simulink library "AFCToolbox2023a"  (R2023a)
settings: Solver=VariableStepAuto  StartTime=0.0  StopTime=10.0  RelTol=1e-3
undefined symbols (not defined in the file or in its folder): AFC5Toolbox_SimuMoudle, AFCToolbox, ax, ay, az, btnSample, C_d, C_dm, C_m, C_t, Control, d, declination_table, dp0, dp1, dp2, dp3, dt, euler_0, g0, I_xyz, inclination_table, J_m, lmd_high, lmd_low, lp_acc_knoise, lp_acc_max, lp_acc_min, lp_acc_seed, lp_GPS_BL_max, lp_GPS_BL_min, lp_GPS_H_max, lp_GPS_H_min, lp_GPS_knoise, lp_GPS_seed, lp_GPS_vel_max, lp_GPS_vel_min, lp_gyro_knoise, lp_gyro_max, lp_gyro_min, lp_gyro_seed, lp_hf_vwind, lp_hs_vwind_interp, lp_kaerorho, lp_kaeroT, lp_kIxyz, lp_kmass, lp_momentx_A0, lp_momentx_Af, lp_momentx_ts, lp_momenty_A0, lp_momenty_Af, lp_momenty_ts, lp_momentz_A0, lp_momentz_Af, lp_momentz_ts, lp_vf_vwind, lp_vs_vwind_interp, lp_vwind_thetax, lp_vwind_thetaz ... (+54)
libraries: $bdroot x104, simulink x75, etargetslib x32, sharedtransform x13, simulink_extras x12, dspstat3 x11, aerolibconvert2 x9, aerolibtransform2 x3, aerolibutil x2, matrix_library x1
(part 4 of 10)

== system AFCToolbox2023a/SimuMoudle/Forces & Moments1/Moments ==
  w_xyz1 : Inport
  w_1234 : Inport  Port=2
  Abs : Abs  SaturateOnIntegerOverflow=off
  Constant : Constant  Value=[1 -1 -1 1;1 1 -1 -1]
  Constant1 : Constant  Value=[1 -1 1 -1]
  Constant2 : Constant  Value=[1 -1 1 -1]
  Constant3 : Constant  Value=[-1 1 -1 1]
  Constant4 : Constant  Value=0
  Disturb : Subsystem
  Dot Product : DotProduct  OutDataTypeStr=Inherit: Inherit via internal rule
  Dot Product1 : DotProduct  OutDataTypeStr=Inherit: Inherit via internal rule
  Dot Product2 : DotProduct  OutDataTypeStr=Inherit: Inherit via internal rule
  Gain : Gain  Gain=C_t
  Gain1 : Gain  Gain=d
  Gain2 : Gain  Gain=C_m
  Gain3 : Gain  Gain=C_dm
  Gain4 : Gain  Gain=-1
  Gain5 : Gain  Gain=J_m
  Gain6 : Gain  Gain=sqrt(2)/2
  M1 : Scope
  Mux : Mux  Inputs=2
  Mux1 : Mux  Inputs=3
  Product : Product  Multiplication=Matrix(*)
  Product{1,3,6..7} (4 alike) : Product
  Scope : Scope
  Selector : Selector  InputPortWidth=3  IndexOptions=Index vector (dialog)  Indices=2  OutputSizes=1
  Selector1 : Selector  InputPortWidth=3  IndexOptions=Index vector (dialog)  Indices=1  OutputSizes=1
  Subtract : Sum  Inputs=3
  Sum of Elements : Sum  Inputs=+
  Sum of Elements1 : Sum  Inputs=+
  M : Outport
  wires:
  Subtract/1 -> Disturb/1(Moment)
  Disturb/1(M) -> M/1, M1/1
  Product1/1 -> Gain2/1, Gain/1
  Gain/1 -> Gain1/1
  Constant/1 -> Gain6/1
  Gain1/1 -> Product/2
  Gain2/1 -> Dot Product2/2
  Constant1/1 -> Dot Product2/1
  Product/1 -> Mux/1
  Dot Product2/1 -> Mux/2
  Abs/1 -> Product3/2
  Product3/1 -> Gain3/1
  w_xyz1/1 -> Abs/1, Product3/1, Selector/1, Selector1/1
  Gain3/1 -> Gain4/1
  Constant2/1 -> Dot Product/1
  Constant3/1 -> Dot Product1/1
  Selector/1 -> Product6/2
  Dot Product/1 -> Sum of Elements/1
  Sum of Elements/1 -> Product6/1
  Dot Product1/1 -> Sum of Elements1/1
  Selector1/1 -> Product7/2
  Sum of Elements1/1 -> Product7/1
  Product6/1 -> Mux1/1
  Product7/1 -> Mux1/2
  Constant4/1 -> Mux1/3
  Mux1/1 -> Gain5/1
  Gain4/1 -> Subtract/1
  Mux/1 -> Subtract/2
  Gain6/1 -> Product/1
  w_1234/1 -> Scope/1, Product1/2, Product1/1, Dot Product1/2, Dot Product/2
  Gain5/1 -> Subtract/3

== system AFCToolbox2023a/SimuMoudle/Forces & Moments1/Parameters ==
  V_xyz : Inport
  xyz : Inport  Port=2
  B to G : Inport  Port=3
  Air Parameter1 : Subsystem
  Gain : Gain  Gain=-1
  Inertia Solution : Subsystem
  Math Function : Math  Operator=transpose  SignedPower=on
  Product : Product  Multiplication=Matrix(*)
  Selector : Selector  InputPortWidth=3  IndexOptions=Index vector (dialog)  Indices=3  OutputSizes=1
  Sum : Sum  Inputs=|+-
  Terminator1 : Terminator
  Terminator2 : Terminator
  Terminator3 : Terminator
  Wind Velocity : Subsystem
  mass P : Subsystem
  modulus of vector : Subsystem  mask(modulus of vector){}
      mask help: solve the modulus of a vector |v|
      mask Display: fprintf('Vector\nModulus')
  Vb_a : Outport
  mass : Outport  Port=2
  Inertia : Outport  Port=3
  g : Outport  Port=4
  wires:
  V_xyz/1 -> Sum/1
  xyz/1 -> Selector/1
  modulus of vector/1(modulus) -> Air Parameter1/1(V)
  Selector/1 -> Air Parameter1/2(h(m)), Wind Velocity/1(height)
  Inertia Solution/1(Inertia) -> Inertia/1
  Wind Velocity/1(V Wind) -> Sum/2
  Sum/1 -> Gain/1, modulus of vector/1(vector)
  Air Parameter1/1(Mach) -> Terminator2/1
  mass P/1(mass) -> mass/1
  Air Parameter1/2(q) -> Terminator1/1
  Air Parameter1/3(Pressure) -> Terminator3/1
  B to G/1 -> Math Function/1
  Math Function/1 -> Product/1
  Product/1 -> Vb_a/1
  Gain/1 -> Product/2
  Air Parameter1/4(g) -> g/1

== system AFCToolbox2023a/SimuMoudle/Forces & Moments1/acc_body ==
  B2G : Inport
  g : Inport  Port=2
  acc_no_g : Inport  Port=3
  Add : Sum
  Constant : Constant  Value=0
  Gain : Gain  Gain=-1
  Mux : Mux  Inputs=3
  Product : Product  Multiplication=Matrix(*)
  Transpose : Math  Operator=transpose  SignedPower=on
  acc : Outport
  wires:
  Gain/1 -> Mux/3
  acc_no_g/1 -> Add/2
  Constant/1 -> Mux/2, Mux/1
  B2G/1 -> Transpose/1
  g/1 -> Gain/1
  Mux/1 -> Add/1
  Add/1 -> Product/2
  Transpose/1 -> Product/1
  Product/1 -> acc/1

== system AFCToolbox2023a/SimuMoudle/LLA2XYZ/LLA2NED ==
  LLA0 : Inport
  LLA : Inport  Port=2
  Angle Conversion2 : aerolibconvert2/Angle Conversion  IU=deg  OU=rad
  Angle Conversion3 : aerolibconvert2/Angle Conversion  IU=deg  OU=rad
  Bus Selector : BusSelector  OutputSignals=lon,lat
  Bus Selector1 : BusSelector  OutputSignals=lat,lon,alt
  Constant1 : Constant  Value=-90
  Constant4 : Constant  Value=0
  Demux : Demux  Outputs=3
  Demux3 : Demux  Outputs=3
  Divide1 : Product  Inputs=**  Multiplication=Matrix(*)
  Gain : Gain  Gain=-1
  Gain1 : Gain  Gain=-1
  LLA to ECEF Position : LLA2ECEF  R=6378137
  LLA to ECEF Position1 : LLA2ECEF  R=6378137
  Mux : Mux  Inputs=3
  Mux2 : Mux  Inputs=3
  Mux5 : Mux  Inputs=2
  Mux6 : Mux  Inputs=2
  Radians to Degrees : simulink_extras/Transformations/Radians to Degrees
  Radians to Degrees1 : simulink_extras/Transformations/Radians to Degrees
  Rotation Angles to Direction Cosine Matrix : sharedtransform/Rotation Angles to Direction Cosine Matrix  rotationOrder=ZYX  aMode=aMode
  Sum : Sum  Inputs=|++
  Sum1 : Sum  Inputs=|+-
  "sensorout " : Outport
  wires:
  Gain1/1 -> Mux/2
  Demux3/2 -> Mux/3  "Yeast"
  Demux3/3 -> Gain1/1
  Demux3/1 -> Mux/1  "Xnorth"
  Radians to Degrees1/1 -> Mux6/2
  Radians to Degrees/1 -> Mux6/1
  LLA/1 -> Demux/1
  Mux/1 -> "sensorout "/1
  Bus Selector1/3 -> LLA to ECEF Position/2  "<alt>"
  Bus Selector1/2 -> Mux5/2  "<lon>"
  Bus Selector1/1 -> Mux5/1  "<lat>"
  Bus Selector/1 -> Angle Conversion2/1  "<lon>"
  Bus Selector/2 -> Gain/1  "<lat>"
  Angle Conversion3/1 -> Mux2/2
  Demux/2 -> Radians to Degrees1/1
  Angle Conversion2/1 -> Mux2/1
  LLA to ECEF Position/1 -> Sum1/2
  Constant1/1 -> Sum/2
  [M_ecef2ned] -> Divide1/1
  Rotation Angles to Direction Cosine Matrix/1 -> [M_ecef2ned]
  Mux2/1 -> Rotation Angles to Direction Cosine Matrix/1
  Demux/1 -> Radians to Degrees/1
  Divide1/1 -> Demux3/1
  [LLA0] -> Bus Selector/1
  [LLA0] -> Bus Selector1/1
  Sum1/1 -> Divide1/2
  Constant4/1 -> Mux2/3
  LLA to ECEF Position1/1 -> Sum1/1
  Gain/1 -> Sum/1
  Mux5/1 -> LLA to ECEF Position/1
  Mux6/1 -> LLA to ECEF Position1/1
  LLA0/1 -> [LLA0]
  Sum/1 -> Angle Conversion3/1
  Demux/3 -> LLA to ECEF Position1/2

== system AFCToolbox2023a/SimuMoudle/Position-Control/Consistent formation control  ==
  u0_k : Inport
  X1_k_1 : Inport  Port=2
  X2_k_1 : Inport  Port=3
  X3_k_1 : Inport  Port=4
  X0_k_1 : Inport  Port=5
  Bus Creator : BusCreator  Inputs=4
  Bus Creator1 : BusCreator  Inputs=3
  Delay5 : Delay  DelayLength=1  InitialCondition=u0
  dp0 : Constant  Value=dp0
  dp1 : Constant  Value=dp1
  dp2 : Constant  Value=dp2
  dp3 : Constant  Value=dp3
  一致性控制——F1 : Subsystem
  一致性控制——F2 : Subsystem
  一致性控制——F3 : Subsystem
  u : Outport
  wires:
  Delay5/1 -> 一致性控制——F2/2(u0_k), 一致性控制——F3/2(u0_k), 一致性控制——F1/1(u0_k)
  Bus Creator1/1 -> u/1
  [u3_k] -> Bus Creator1/3  "u3_k"
  [u2_k] -> Bus Creator1/2  "u2_k"
  [u1_k] -> Bus Creator1/1  "u1_k"
  一致性控制——F3/1(u3_k) -> [u3_k]
  一致性控制——F2/1(u2_k) -> [u2_k]
  [dp] -> 一致性控制——F1/5(dp), 一致性控制——F2/1(dp), 一致性控制——F3/1(dp)
  一致性控制——F1/1(u1_k) -> [u1_k]
  X2_k_1/1 -> 一致性控制——F1/4(X2_k_1), 一致性控制——F3/5(X2_k_1), 一致性控制——F2/5(X2_k_1)
  X1_k_1/1 -> 一致性控制——F3/4(X1_k_1), 一致性控制——F2/4(X1_k_1), 一致性控制——F1/3(X1_k_1)
  X0_k_1/1 -> 一致性控制——F3/3(X0_k_1), 一致性控制——F2/3(X0_k_1), 一致性控制——F1/2(X0_k_1)
  u0_k/1 -> Delay5/1
  Bus Creator/1 -> [dp]
  dp3/1 -> Bus Creator/4  "dp3"
  dp2/1 -> Bus Creator/3  "dp2"
  dp1/1 -> Bus Creator/2  "dp1"
  dp0/1 -> Bus Creator/1  "dp0"
  X3_k_1/1 -> 一致性控制——F3/6(X3_k_1), 一致性控制——F2/6(X3_k_1)

== system AFCToolbox2023a/SimuMoudle/Position-Control/Leader ==
  note: Leader加速度
  Add{,1..3} (4 alike) : Sum
  Add4 : Sum  Inputs=+-
  Bus Creator : BusCreator  Inputs=6
  Delay : Delay  DelayLength=1  InitialCondition=theta0
  Delay1 : Delay  DelayLength=1  InitialCondition=phi0
  Delay2 : Delay  DelayLength=1  InitialCondition=v0
  Delay3 : Delay  DelayLength=1  InitialCondition=p0
  Delay4 : Delay  DelayLength=1  InitialCondition=p0
  Gain1 : Gain  Gain=1/dt
  Gain{2..5} (4 alike) : Gain  Gain=dt
  MATLAB Function : MATLAB Function  TreatAsAtomicUnit=on
  Mux : Mux  Inputs=3
  Product : Product  Multiplication=Matrix(*)
  Reshape : Reshape  OutputDimensionality=Customize  OutputDimensions=[3,1]
  Scope : Scope  NumInputPorts=2
  Subsystem : Subsystem
  Transpose : Math  Operator=transpose
  W0-Φ : Subsystem
  r0-v : Subsystem
  w0-θ : Subsystem
  质心运动方程 : Subsystem
  p0_k : Outport
  u0_k——xyz加速度 : Outport  Port=2
  X0_k_1 : Outport  Port=3
  v0_k : Outport  Port=4
  w0_k : Outport  Port=5
  W0_k : Outport  Port=6
  wires:
  Delay4/1 -> Add4/2
  Gain1/1 -> Scope/2
  Add4/1 -> Gain1/1
  Transpose/1 -> u0_k——xyz加速度/1
  Product/1 -> Transpose/1
  质心运动方程/1(v000) -> Gain2/1, Scope/1, [v000_k_1]
  [p0_k_1] -> Bus Creator/6  "p0_k_1"
  [v000_k_1] -> Bus Creator/5  "v000_k_1"
  Bus Creator/1 -> X0_k_1/1
  [rwW0_k] -> Bus Creator/1  "rwW0_k"
  [v0_k_1] -> Bus Creator/4  "v0_k_1"
  [phi0_k_1] -> Bus Creator/3  "phi0_k_1"
  [theta0_k_1] -> Bus Creator/2  "theta0_k_1"
  [v0_k_1] -> MATLAB Function/3(v)
  [phi0_k_1] -> MATLAB Function/2(phi)
  [theta0_k_1] -> MATLAB Function/1(theta)
  Reshape/1 -> Product/2, [rwW0_k]
  W0-Φ/1(W0) -> Mux/3, W0_k/1, Gain5/1
  Gain4/1 -> Add1/2
  Gain3/1 -> Add2/2
  Delay3/1 -> Add3/1, Delay4/1, [p0_k_1]
  Add3/1 -> p0_k/1, Add4/1, Delay3/1
  Gain2/1 -> Add3/2
  Delay2/1 -> [v0_k_1], Add2/1
  Add2/1 -> v0_k/1, 质心运动方程/3(v0), Delay2/1
  r0-v/1(r0) -> Mux/1, Gain3/1
  Add1/1 -> 质心运动方程/2(phi0), Delay1/1
  Delay1/1 -> [phi0_k_1], Add1/1
  w0-θ/1(w0) -> Mux/2, w0_k/1, Gain4/1
  Delay/1 -> Add/1, [theta0_k_1]
  Add/1 -> 质心运动方程/1(theta0), Delay/1
  Gain5/1 -> Add/2
  Mux/1 -> Reshape/1
  MATLAB Function/1(J) -> Product/1

== system AFCToolbox2023a/SimuMoudle/SimuBaro/Baro model ==
  H : Inport
  MATLAB Function : MATLAB Function  TreatAsAtomicUnit=on
  MATLAB Function1 : MATLAB Function  TreatAsAtomicUnit=on
  Scope : Scope  NumInputPorts=2
  Scope1 : Scope
  Selector : Selector  InputPortWidth=3  IndexOptions=Index vector (dialog)  Indices=[3]  OutputSizes=1
  Zero-Order Hold3 : ZeroOrderHold  SampleTime=lp_GPS_sample_time
  bias & noise z : Subsystem  mask(Bias and Noise Model){noise_min=lp_GPS_H_min, noise_max=lp_GPS_H_max, noise_seed=lp_GPS_seed, noise_k=lp_GPS_knoise, sample_time=lp_GPS_sample_time}
      mask prompts: noise_min "Minimum of the noise:"; noise_max "Maximum of the noise:"; noise_seed "Seed of the noise:"; noise_k "Noise coefficiet:"; sample_time "Sample time"
  Pa out : Outport
  Tem out : Outport  Port=2
  wires:
  MATLAB Function1/2(temperature) -> Scope1/1, Tem out/1
  MATLAB Function1/1(pressure) -> Scope/2, Pa out/1
  Selector/1 -> Zero-Order Hold3/1
  MATLAB Function/1(P) -> Scope/1
  bias & noise z/1(real) -> MATLAB Function/1(h), MATLAB Function1/1(altitude)
  H/1 -> Selector/1
  Zero-Order Hold3/1 -> bias & noise z/1(normal)

== system AFCToolbox2023a/SimuMoudle/SimuComOut_BytePack/CheckSum ==
  In1 : Inport
  Add : Sum
  Bitwise Operator : simulink/Logic and Bit Operations/Bitwise Operator  logicop=NOT  UseBitMask=off  BitMask=bin2dec('11011001')  BitMaskRealWorld=Stored Integer
  Bitwise OR : simulink/Logic and Bit Operations/Bitwise Operator  logicop=AND  UseBitMask=on  BitMask=hex2dec('FF')  BitMaskRealWorld=Stored Integer
  Constant : Constant
  Data Type Conversion : DataTypeConversion  OutDataTypeStr=uint16  SaturateOnIntegerOverflow=off  RndMeth=Floor
  Data Type Conversion1 : DataTypeConversion  OutDataTypeStr=uint8  SaturateOnIntegerOverflow=off  RndMeth=Floor
  Data Type Conversion2 : DataTypeConversion  OutDataTypeStr=uint8  SaturateOnIntegerOverflow=off  RndMeth=Floor
  Data Type Conversion3 : DataTypeConversion  OutDataTypeStr=uint8  SaturateOnIntegerOverflow=off  RndMeth=Floor
  Sum of Elements : Sum  Inputs=+
  Out1 : Outport
  wires:
  Data Type Conversion3/1 -> Out1/1
  Sum of Elements/1 -> Bitwise OR/1
  Bitwise OR/1 -> Data Type Conversion1/1
  Data Type Conversion/1 -> Sum of Elements/1
  Data Type Conversion1/1 -> Bitwise Operator/1
  In1/1 -> Data Type Conversion/1
  Bitwise Operator/1 -> Add/1
  Constant/1 -> Data Type Conversion2/1
  Data Type Conversion2/1 -> Add/2
  Add/1 -> Data Type Conversion3/1

== system AFCToolbox2023a/SimuMoudle/SimuGps/LLA model ==
  xyz : Inport
  Demux : Demux  Outputs=3
  Mux : Mux  Inputs=3
  Subsystem1 : Subsystem
  Zero-Order Hold1 : ZeroOrderHold  SampleTime=lp_GPS_sample_time
  Zero-Order Hold2 : ZeroOrderHold  SampleTime=lp_GPS_sample_time
  Zero-Order Hold3 : ZeroOrderHold  SampleTime=lp_GPS_sample_time
  bias & noise x : Subsystem  mask(Bias and Noise Model){noise_min=lp_GPS_BL_min, noise_max=lp_GPS_BL_max, noise_seed=lp_GPS_seed, noise_k=lp_GPS_knoise, sample_time=lp_GPS_sample_time}
      mask prompts: noise_min "Minimum of the noise:"; noise_max "Maximum of the noise:"; noise_seed "Seed of the noise:"; noise_k "Noise coefficiet:"; sample_time "Sample time"
  bias & noise x2 : Subsystem  mask(Bias and Noise Model){noise_min=lp_GPS_BL_min, noise_max=lp_GPS_BL_max, noise_seed=lp_GPS_seed, noise_k=lp_GPS_knoise, sample_time=lp_GPS_sample_time}
      mask prompts: noise_min "Minimum of the noise:"; noise_max "Maximum of the noise:"; noise_seed "Seed of the noise:"; noise_k "Noise coefficiet:"; sample_time "Sample time"
  bias & noise z : Subsystem  mask(Bias and Noise Model){noise_min=lp_GPS_H_min, noise_max=lp_GPS_H_max, noise_seed=lp_GPS_seed, noise_k=lp_GPS_knoise, sample_time=lp_GPS_sample_time}
      mask prompts: noise_min "Minimum of the noise:"; noise_max "Maximum of the noise:"; noise_seed "Seed of the noise:"; noise_k "Noise coefficiet:"; sample_time "Sample time"
  LLA out : Outport
  wires:
  Subsystem1/1(LLA) -> LLA out/1
  bias & noise z/1(real) -> Mux/3, Subsystem1/3(Z)
  bias & noise x2/1(real) -> Mux/2, Subsystem1/2(Y)
  bias & noise x/1(real) -> Mux/1, Subsystem1/1(X)
  Zero-Order Hold1/1 -> bias & noise x/1(normal)
  Zero-Order Hold2/1 -> bias & noise x2/1(normal)
  Zero-Order Hold3/1 -> bias & noise z/1(normal)
  xyz/1 -> Demux/1
  Demux/1 -> Zero-Order Hold1/1
  Demux/2 -> Zero-Order Hold2/1
  Demux/3 -> Zero-Order Hold3/1

== system AFCToolbox2023a/SimuMoudle/SimuGps/Vel model ==
  Vel_GPS : Inport
  Add : Sum
  Atan2 : Trigonometry  Operator=atan2
  Demux : Demux  Outputs=3
  Gain1 : Gain  Gain=-1
  Mux : Mux  Inputs=3
  Radians to Degrees : simulink_extras/Transformations/Radians to Degrees
  Scope : Scope
  Sqrt : Sqrt
  Square : Math  Operator=square
  Square1 : Math  Operator=square
  Zero-Order Hold : ZeroOrderHold  SampleTime=lp_GPS_sample_time
  Zero-Order Hold1 : ZeroOrderHold  SampleTime=lp_GPS_sample_time
  Zero-Order Hold2 : ZeroOrderHold  SampleTime=lp_GPS_sample_time
  bias & noise x : Subsystem  mask(Bias and Noise Model){noise_min=lp_GPS_vel_min, noise_max=lp_GPS_vel_max, noise_seed=lp_GPS_seed, noise_k=lp_GPS_knoise, sample_time=lp_GPS_sample_time}
      mask prompts: noise_min "Minimum of the noise:"; noise_max "Maximum of the noise:"; noise_seed "Seed of the noise:"; noise_k "Noise coefficiet:"
  bias & noise x1 : Subsystem  mask(Bias and Noise Model){noise_min=lp_GPS_vel_min, noise_max=lp_GPS_vel_max, noise_seed=lp_GPS_seed, noise_k=lp_GPS_knoise, sample_time=lp_GPS_sample_time}
      mask prompts: noise_min "Minimum of the noise:"; noise_max "Maximum of the noise:"; noise_seed "Seed of the noise:"; noise_k "Noise coefficiet:"
  bias & noise x3 : Subsystem  mask(Bias and Noise Model){noise_min=lp_GPS_vel_min, noise_max=lp_GPS_vel_max, noise_seed=lp_GPS_seed, noise_k=lp_GPS_knoise, sample_time=lp_GPS_sample_time}
      mask prompts: noise_min "Minimum of the noise:"; noise_max "Maximum of the noise:"; noise_seed "Seed of the noise:"; noise_k "Noise coefficiet:"
  Vel_GPS out : Outport
  Vg_地速 : Outport  Port=2
  Psi_GPS_航向角 : Outport  Port=3
  wires:
  Sqrt/1 -> Vg_地速/1
  Add/1 -> Sqrt/1
  Square1/1 -> Add/2
  Square/1 -> Add/1
  bias & noise x/1(real) -> Mux/1, Atan2/2, Square/1
  Gain1/1 -> Psi_GPS_航向角/1
  Atan2/1 -> Radians to Degrees/1, Gain1/1
  Radians to Degrees/1 -> Scope/1
  Mux/1 -> Vel_GPS out/1
  Zero-Order Hold1/1 -> bias & noise x3/1(normal)
  Zero-Order Hold/1 -> bias & noise x/1(normal)
  Vel_GPS/1 -> Demux/1
  Zero-Order Hold2/1 -> bias & noise x1/1(normal)
  Demux/1 -> Zero-Order Hold/1
  Demux/2 -> Zero-Order Hold1/1
  Demux/3 -> Zero-Order Hold2/1
  bias & noise x1/1(real) -> Mux/3
  bias & noise x3/1(real) -> Mux/2, Atan2/1, Square1/1

== system AFCToolbox2023a/SimuMoudle/SimuICM/acclerate  model2 ==
  axyz : Inport
  Demux : Demux  Outputs=3
  Mux : Mux  Inputs=3
  Mux1 : Mux  Inputs=3
  Subsystem : Subsystem
  Subsystem1 : Subsystem
  Subsystem2 : Subsystem
  bias & noise x : Subsystem  mask(Bias and Noise Model){noise_min=lp_gyro_min, noise_max=lp_gyro_max, noise_seed=lp_gyro_seed, noise_k=lp_gyro_knoise}
      mask prompts: noise_min "Minimum of the noise:"; noise_max "Maximum of the noise:"; noise_seed "Seed of the noise:"; noise_k "Noise coefficiet:"
  bias & noise y : Subsystem  mask(Bias and Noise Model){noise_min=lp_gyro_min, noise_max=lp_gyro_max, noise_seed=lp_gyro_seed, noise_k=lp_gyro_knoise}
      mask prompts: noise_min "Minimum of the noise:"; noise_max "Maximum of the noise:"; noise_seed "Seed of the noise:"; noise_k "Noise coefficiet:"
  bias & noise z : Subsystem  mask(Bias and Noise Model){noise_min=lp_gyro_min, noise_max=lp_gyro_max, noise_seed=lp_gyro_seed, noise_k=lp_gyro_knoise}
      mask prompts: noise_min "Minimum of the noise:"; noise_max "Maximum of the noise:"; noise_seed "Seed of the noise:"; noise_k "Noise coefficiet:"
  accel out : Outport
  wires:
  Subsystem2/1(real) -> Mux1/3
  Subsystem1/1(real) -> Mux1/2
  Subsystem/1(real) -> Mux1/1
  Demux/1 -> Subsystem/1(normal), bias & noise x/1(normal)
  axyz/1 -> Demux/1
  bias & noise x/1(real) -> Mux/1
  Demux/2 -> Subsystem1/1(normal), bias & noise y/1(normal)
  Demux/3 -> Subsystem2/1(normal), bias & noise z/1(normal)
  bias & noise y/1(real) -> Mux/2
  bias & noise z/1(real) -> Mux/3
  Mux1/1 -> accel out/1

== system AFCToolbox2023a/SimuMoudle/SimuICM/gyro model1 ==
  wxyz : Inport
  Demux : Demux  Outputs=3
  Mux : Mux  Inputs=3
  Mux1 : Mux  Inputs=3
  Subsystem : Subsystem
  Subsystem1 : Subsystem
  Subsystem2 : Subsystem
  bias & noise x : Subsystem  mask(Bias and Noise Model){noise_min=lp_gyro_min, noise_max=lp_gyro_max, noise_seed=lp_gyro_seed, noise_k=lp_gyro_knoise}
      mask prompts: noise_min "Minimum of the noise:"; noise_max "Maximum of the noise:"; noise_seed "Seed of the noise:"; noise_k "Noise coefficiet:"
  bias & noise y : Subsystem  mask(Bias and Noise Model){noise_min=lp_gyro_min, noise_max=lp_gyro_max, noise_seed=lp_gyro_seed, noise_k=lp_gyro_knoise}
      mask prompts: noise_min "Minimum of the noise:"; noise_max "Maximum of the noise:"; noise_seed "Seed of the noise:"; noise_k "Noise coefficiet:"
  bias & noise z : Subsystem  mask(Bias and Noise Model){noise_min=lp_gyro_min, noise_max=lp_gyro_max, noise_seed=lp_gyro_seed, noise_k=lp_gyro_knoise}
      mask prompts: noise_min "Minimum of the noise:"; noise_max "Maximum of the noise:"; noise_seed "Seed of the noise:"; noise_k "Noise coefficiet:"
  gyro out : Outport
  wires:
  bias & noise z/1(real) -> Mux/3
  bias & noise y/1(real) -> Mux/2
  Demux/3 -> Subsystem2/1(normal), bias & noise z/1(normal)
  Demux/2 -> bias & noise y/1(normal), Subsystem1/1(normal)
  bias & noise x/1(real) -> Mux/1
  wxyz/1 -> Demux/1
  Demux/1 -> bias & noise x/1(normal), Subsystem/1(normal)
  Subsystem/1(real) -> Mux1/1
  Subsystem1/1(real) -> Mux1/2
  Subsystem2/1(real) -> Mux1/3
  Mux1/1 -> gyro out/1

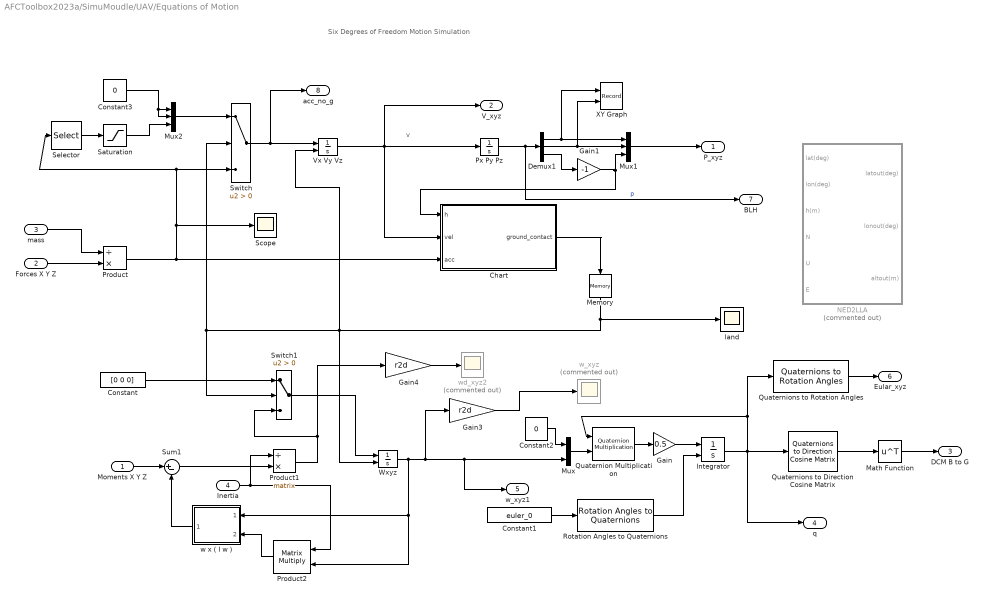
== system AFCToolbox2023a/SimuMoudle/UAV/Equations of Motion ==
  note: Six Degrees of Freedom Motion Simulation
  note: v
  Moments X Y Z : Inport
  Forces X Y Z : Inport  Port=2
  mass : Inport  Port=3
  Inertia : Inport  Port=4
  Chart : Stateflow chart  TreatAsAtomicUnit=on
  Constant : Constant  Value=[0 0 0]
  Constant1 : Constant  Value=euler_0
  Constant2 : Constant  Value=0
  Constant3 : Constant  Value=0
  Demux1 : Demux  Outputs=3
  Gain : Gain  Gain=0.5
  Gain1 : Gain  Gain=-1
  Gain3 : Gain  Gain=r2d
  Gain4 : Gain  Gain=r2d
  Integrator : Integrator  InitialConditionSource=external  InitialCondition=[1 0 0 0]
  Math Function : Math  Operator=transpose  SignedPower=on
  Memory : Memory
  Mux : Mux  Inputs=2
  Mux1 : Mux  Inputs=3
  Mux2 : Mux  Inputs=3
  NED2LLA : Subsystem  Commented=on
  Product : Product  Inputs=/*  RndMeth=Zero
  Product1 : Product  Inputs=/*  Multiplication=Matrix(*)  RndMeth=Zero
  Product2 : Product  Multiplication=Matrix(*)  RndMeth=Zero
  Px Py Pz : Integrator  InitialCondition=[0,0,0]
  Quaternion Multiplication : aerolibutil/Quaternion Multiplication
  Quaternions to Direction Cosine Matrix : sharedtransform/Quaternions to  Direction Cosine Matrix  aMode=aMode
  Quaternions to Rotation Angles : sharedtransform/Quaternions to Rotation Angles  rotationOrder=ZYX  aMode=aMode
  Rotation Angles to Quaternions : sharedtransform/Rotation Angles to Quaternions  rotationOrder=ZYX  aMode=aMode
  Saturation : Saturate  UpperLimit=0  LowerLimit=-inf
  Scope : Scope
  Selector : Selector  InputPortWidth=3  IndexOptions=Index vector (dialog)  Indices=[3]  OutputSizes=1
  Sum1 : Sum  Inputs=|+-
  Switch : Switch  Criteria=u2 > Threshold  SaturateOnIntegerOverflow=off  InputSameDT=off
  Switch1 : Switch  Criteria=u2 > Threshold  SaturateOnIntegerOverflow=off  InputSameDT=off
  Vx Vy Vz : Integrator  ExternalReset=level  InitialCondition=velocity_0
  Wxyz : Integrator  ExternalReset=level  InitialCondition=omega_0
  XY Graph : Record  FileSettingsInternal="{\"entries\":[{\"content\":{\"excelSettings\":{\"content\":{},\"type\":\"Streamout.ExcelSettings\"},\"parquetSettings\":{\"content\":{},\"type\":\"Streamout.ParquetSettings\"}},\"type\":\"Streamout.FileSettingStorage\",\"uuid\":\"\"}],\"packageUris\":[\"http:\\/\\/schema.mathworks.com\\/mf0\\/streamout_blocks\\/R2020a\"],\"version\":\"1.0\"}"  Layout=[1 1]  SignalsInternal="{\"entries\":[{\"content\":{},\"type\":\"RecordBlkView.InputSignals\",\"uuid\":\"\"}],\"packageUris\":[\"http:\\/\\/schema.mathworks.com\\/mf0\\/streamout_blocks\\/R2020a\"],\"version\":\"1.0\"}"  VisualizationBindings="{\"sparklinesplugin\":{\"info\":[{\"bindingParametersList\":[],\"subplotID\":1}]}}"  CompatibilityTag=XY  st=-1
  land : Scope
  w x ( I w ) : Subsystem  mask(Cross Product){}
      mask help: [a;b;c] x [x;y;z] = [bz-cy; cx-az; ay-bx]
      mask Display: fprintf('Cross\nProduct')
  w_xyz : Scope  Commented=on
  wd_xyz2 : Scope  Commented=on
  P_xyz : Outport  InitialOutput=0
  V_xyz : Outport  Port=2  InitialOutput=0
  DCM B to G : Outport  Port=3  InitialOutput=0
  q : Outport  Port=4  InitialOutput=0
  w_xyz1 : Outport  Port=5  InitialOutput=0
  Eular_xyz : Outport  Port=6  InitialOutput=0
  BLH : Outport  Port=7  InitialOutput=0
  acc_no_g : Outport  Port=8  InitialOutput=0
  wires:
  Product2/1 -> w x ( I w )/2(b(1) b(2) b(3))
  Inertia/1 -> Product2/1, Product1/1
  Sum1/1 -> Product1/2
  Forces X Y Z/1 -> Product/2
  mass/1 -> Product/1
  Product1/1 -> Gain4/1, Switch1/3
  Quaternions to Direction Cosine Matrix/1 -> Math Function/1
  Gain3/1 -> w_xyz/1
  Gain4/1 -> wd_xyz2/1
  w x ( I w )/1(c(1) c(2) c(3)) -> Sum1/2
  Vx Vy Vz/1 -> Chart/2(vel), Px Py Pz/1, V_xyz/1
  Wxyz/1 -> w x ( I w )/1(a(1) a(2) a(3)), Product2/2, Gain3/1, w_xyz1/1, Mux/2
  Moments X Y Z/1 -> Sum1/1
  Constant2/1 -> Mux/1
  Mux/1 -> Quaternion Multiplication/2
  Quaternion Multiplication/1 -> Gain/1
  Gain/1 -> Integrator/1
  Rotation Angles to Quaternions/1 -> Integrator/2
  Constant1/1 -> Rotation Angles to Quaternions/1
  Quaternions to Rotation Angles/1 -> Eular_xyz/1
  Demux1/1 -> XY Graph/1, Mux1/1
  Demux1/2 -> XY Graph/2, Mux1/2
  Gain1/1 -> Mux1/3, Chart/1(h)
  Demux1/3 -> Gain1/1
  Px Py Pz/1 -> BLH/1, Demux1/1  "p"
  Product/1 -> Scope/1, Selector/1, Switch/3, Chart/3(acc)
  Chart/1(ground_contact) -> Memory/1
  Memory/1 -> Wxyz/2, Switch1/2, Switch/2, Vx Vy Vz/2, land/1
  Constant3/1 -> Mux2/2, Mux2/1
  Selector/1 -> Saturation/1
  Saturation/1 -> Mux2/3
  Mux2/1 -> Switch/1
  Switch/1 -> acc_no_g/1, Vx Vy Vz/1
  Constant/1 -> Switch1/1
  Math Function/1 -> DCM B to G/1
  Integrator/1 -> Quaternions to Direction Cosine Matrix/1, Quaternion Multiplication/1, Quaternions to Rotation Angles/1, q/1
  Switch1/1 -> Wxyz/1
  Mux1/1 -> P_xyz/1

== system AFCToolbox2023a/SimuMoudle/UAV/Forces & Moments ==
  acc_no_g : Inport
  B to G : Inport  Port=2
  V_xyz : Inport  Port=3
  w1234 : Inport  Port=4
  xyz : Inport  Port=5
  w_xyz1 : Inport  Port=6
  Forces : Subsystem
  Moments : Subsystem
  Parameters : Subsystem
      mask init:
      | % port_label('input', 1, '\delta_x_ _c \delta_y_ _c \delta_z_ _c','texmode','on')
      | % port_label('output', 1, '\delta_x \delta_y \delta_z','texmode','on')
  acc_body : Subsystem
  F : Outport
  M : Outport  Port=2
  mass : Outport  Port=3
  Inertia : Outport  Port=4
  acc : Outport  Port=5
  wires:
  Forces/1("F ") -> F/1
  Moments/1(M) -> M/1
  xyz/1 -> Parameters/2(xyz)
  V_xyz/1 -> Parameters/1(V_xyz)
  w_xyz1/1 -> Moments/1(w_xyz1)
  Parameters/2(mass) -> mass/1, Forces/4(mass)
  Parameters/1(Vb_a) -> Forces/3(Vb_a)
  w1234/1 -> Moments/2(w_1234), Forces/2(w1234)
  B to G/1 -> acc_body/1(B2G), Forces/1(B to G), Parameters/3(B to G)
  Parameters/4(g) -> acc_body/2(g), Forces/5(g)
  Parameters/3(Inertia) -> Inertia/1
  acc_no_g/1 -> acc_body/3(acc_no_g)
  acc_body/1(acc) -> acc/1

== system AFCToolbox2023a/SimuMoudle/UAV/Subsystem3 ==
  Pos : Inport
  Demux1 : Demux  Outputs=3
  Gain1 : Gain  Gain=-1
  Mux1 : Mux  Inputs=3
  Out1 : Outport
  wires:
  Pos/1 -> Demux1/1
  Demux1/1 -> Mux1/1
  Demux1/3 -> Gain1/1
  Mux1/1 -> Out1/1
  Demux1/2 -> Mux1/2
  Gain1/1 -> Mux1/3

== system AFCToolbox2023a/TEST MOUDLE/TEST AD//IV/Subsystem3 ==
  Input : Inport
  Enable : EnablePort
  Constant : Constant  Value=0.42
  Gain1 : Gain  Gain=6.339
  Sum1 : Sum  Inputs=|++
  1 : Outport
  wires:
  Gain1/1 -> Sum1/1
  Sum1/1 -> 1/1
  Constant/1 -> Sum1/2
  Input/1 -> Gain1/1

== system AFCToolbox2023a/TEST MOUDLE/TEST POD IN/Subsystem1 ==
  In1 : Inport
  Add : Sum
  Bitwise Operator : simulink/Logic and Bit Operations/Bitwise Operator  logicop=NOT  UseBitMask=off  BitMask=bin2dec('11011001')  BitMaskRealWorld=Stored Integer
  Bitwise OR : simulink/Logic and Bit Operations/Bitwise Operator  logicop=AND  UseBitMask=on  BitMask=hex2dec('FF')  BitMaskRealWorld=Stored Integer
  Constant : Constant
  Data Type Conversion : DataTypeConversion  OutDataTypeStr=uint16  SaturateOnIntegerOverflow=off  RndMeth=Floor
  Data Type Conversion1 : DataTypeConversion  OutDataTypeStr=uint8  SaturateOnIntegerOverflow=off  RndMeth=Floor
  Data Type Conversion2 : DataTypeConversion  OutDataTypeStr=uint16  SaturateOnIntegerOverflow=off  RndMeth=Floor
  Data Type Conversion3 : DataTypeConversion  OutDataTypeStr=uint8  SaturateOnIntegerOverflow=off  RndMeth=Floor
  Data Type Conversion4 : DataTypeConversion  OutDataTypeStr=uint16  SaturateOnIntegerOverflow=off  RndMeth=Floor
  Sum of Elements : Sum  Inputs=+
  Out1 : Outport
  wires:
  Data Type Conversion3/1 -> Out1/1
  Sum of Elements/1 -> Bitwise OR/1
  Bitwise OR/1 -> Data Type Conversion1/1
  Data Type Conversion/1 -> Sum of Elements/1
  Data Type Conversion1/1 -> Bitwise Operator/1
  In1/1 -> Data Type Conversion/1
  Bitwise Operator/1 -> Data Type Conversion4/1
  Constant/1 -> Data Type Conversion2/1
  Data Type Conversion2/1 -> Add/2
  Add/1 -> Data Type Conversion3/1
  Data Type Conversion4/1 -> Add/1

== system AFCToolbox2023a/基础导航算法模型库/ECL EKF/Bias Eliminate2 ==
  gyro_B_rad/s_ori : Inport
  Digital Clock : DigitalClock
  Memory : Memory
  Scope : Scope  NumInputPorts=2
  Subsystem : Subsystem
  Sum : Sum  Inputs=|+-
  Switch : Switch  Criteria=u2 > Threshold  Threshold=1.5  SaturateOnIntegerOverflow=off  InputSameDT=off
  Out1 : Outport
  wires:
  gyro_B_rad/s_ori/1 -> Subsystem/1(data), Scope/2, Sum/1
  Sum/1 -> Out1/1
  Digital Clock/1 -> Switch/2
  Subsystem/1(mean_data) -> Switch/3
  Switch/1 -> Scope/1, Sum/2, Memory/1
  Memory/1 -> Switch/1

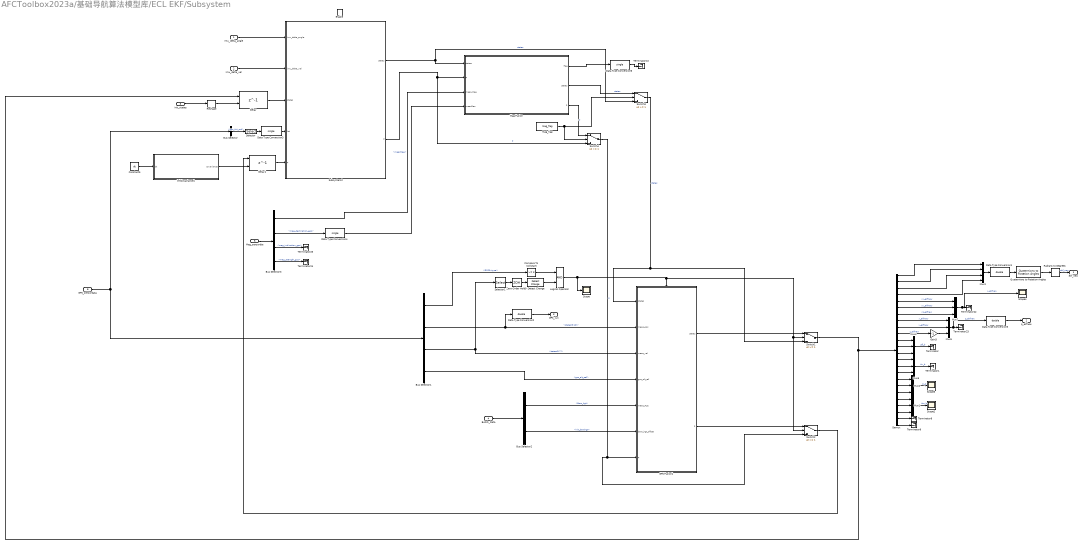
== system AFCToolbox2023a/基础导航算法模型库/ECL EKF/Subsystem ==
  imu_delta_angle : Inport
  imu_delta_vel : Inport  Port=2
  init_states : Inport  Port=3
  BARO_Data : Inport  Port=4
  Mag_sensordta : Inport  Port=5
  GPS_sensordata : Inport  Port=6
  Enable : EnablePort
  Bus Selector : BusSelector  OutputSignals=gps_LLA_rad
  Bus Selector1 : BusSelector  OutputSignals=GPSfixtype,states(8:10),states(5:7),gps_alt_aef
  Bus Selector2 : BusSelector  OutputSignals=Baro_hgt,init_barohgt
  Bus Selector3 : BusSelector  OutputSignals=measMag,mag_declination_gps,mag_inclination_gps,mag_strength_gps
  Compare To Constant : simulink/Logic and Bit Operations/Compare To Constant  relop=>=  const=3  OutDataTypeStr=boolean
  Constant5 : Constant  Value=dt  OutDataTypeStr=single
  Data Type Conversion1 : DataTypeConversion  OutDataTypeStr=double  SaturateOnIntegerOverflow=off  RndMeth=Floor
  Data Type Conversion2 : DataTypeConversion  OutDataTypeStr=double  SaturateOnIntegerOverflow=off  RndMeth=Floor
  Data Type Conversion3 : DataTypeConversion  OutDataTypeStr=single  SaturateOnIntegerOverflow=off  RndMeth=Floor
  Data Type Conversion4 : DataTypeConversion  OutDataTypeStr=single  SaturateOnIntegerOverflow=off  RndMeth=Floor
  Data Type Conversion5 : DataTypeConversion  OutDataTypeStr=double  SaturateOnIntegerOverflow=off  RndMeth=Floor
  Data Type Conversion6 : DataTypeConversion  OutDataTypeStr=single  SaturateOnIntegerOverflow=off  RndMeth=Floor
  Delay : Delay  DelayLength=1  InitialConditionSource=Input port  InitialCondition=0  UseCircularBuffer=on
      settings: InputPortMap=u0,p4
  Delay1 : Delay  DelayLength=1  InitialConditionSource=Input port  InitialCondition=0  UseCircularBuffer=on
      settings: InputPortMap=u0,p4
  Demux : Demux  Outputs=24
  Detect Change : simulink/Logic and Bit Operations/Detect Change  vinit=0  OutDataTypeStr=boolean
  GPS Fusion1 : Subsystem
  Gain3 : Gain  Gain=-1
  InitCovariance1 : MATLAB Function  TreatAsAtomicUnit=on
  Logical Operator : Logic  AllPortsSameDT=off  OutDataTypeStr=boolean
  Mag Fusion : Subsystem
  Mux{1..2,4..7} (6 alike) : Mux  Inputs=3
  Mux3 : Mux
  Quaternions to Rotation Angles : sharedtransform/Quaternions to Rotation Angles  rotationOrder=ZYX  aMode=aMode
  Radians to Degrees : simulink_extras/Transformations/Radians to Degrees
  Reshape : Reshape  OutputDimensionality=Customize  OutputDimensions=[24,1]
  Scope{,2..4} (4 alike) : Scope
  Selector : Selector  InputPortWidth=3  IndexOptions=Index vector (dialog)  Indices=[1]  OutputSizes=1
  Selector1 : Selector  InputPortWidth=3  IndexOptions=Index vector (dialog)  Indices=[1]  OutputSizes=1
  Subsystem2 : Subsystem
  Switch{1..4} (4 alike) : Switch  Threshold=1  OutDataTypeStr=single  SaturateOnIntegerOverflow=off  InputSameDT=off
  Terminator{,1,8..10,22..25} (9 alike) : Terminator
  Zero-Order Hold9 : ZeroOrderHold  SampleTime=-1
  mag_flag : Constant  Value=mag_flag
  ekf_new : Outport
  p_ekfnew : Outport  Port=2
  GPS_xyz : Outport  Port=3
  wires:
  mag_flag/1 -> Switch3/2, Switch4/2
  Mag Fusion/3(P) -> Switch4/1  "P"
  Mag Fusion/2(states) -> Switch3/1  "states"
  Switch4/1 -> GPS Fusion1/7("P "), Switch2/3  "P"
  Switch3/1 -> Switch1/3, GPS Fusion1/1("states ")  "states"
  Subsystem2/1(states) -> Mag Fusion/1("states "), Switch3/3  "states"
  Subsystem2/2(P) -> Mag Fusion/2("P "), Switch4/3  "P"
  Data Type Conversion6/1 -> Terminator10/1
  Data Type Conversion4/1 -> Mag Fusion/4(measDec)
  Data Type Conversion3/1 -> Subsystem2/4(lat)
  Mux2/1 -> Scope3/1  "m_b"
  Mux1/1 -> Scope2/1  "Δm_b"
  Delay1/1 -> Subsystem2/5("P ")
  InitCovariance1/1(covariance) -> Delay1/2
  Demux/16 -> Mux5/3
  Bus Selector1/1 -> Compare To Constant/1  "<GPSfixtype>"
  Mux4/1 -> Terminator/1  "Δθ_b"
  Delay/1 -> Subsystem2/3("states ")
  Compare To Constant/1 -> Logical Operator/1
  Logical Operator/1 -> GPS Fusion1/Enable, Switch2/2, Switch1/2, Scope/1
  Bus Selector1/2 -> Data Type Conversion2/1, GPS Fusion1/2(meas_pos)  "<states(8:10)>"
  Bus Selector3/3 -> Terminator25/1  "<mag_inclination_gps>"
  Quaternions to Rotation Angles/1 -> Radians to Degrees/1
  GPS_sensordata/1 -> Bus Selector/1, Bus Selector1/1
  Switch1/1 -> Demux/1, Delay/1
  Gain3/1 -> Mux6/3
  GPS Fusion1/2(P) -> Switch2/1
  Demux/2 -> Mux3/2
  Demux/20 -> Mux1/1
  Demux/10 -> Gain3/1  "z_ekfnew"
  Detect Change/1 -> Logical Operator/2
  Demux/9 -> Mux6/2  "y_ekfnew"
  Demux/14 -> Mux5/1
  Reshape/1 -> Delay/2
  Bus Selector3/1 -> Mag Fusion/3(meas_Mag)  "<measMag>"
  Constant5/1 -> InitCovariance1/1(dt)
  Demux/19 -> Mux2/3
  Demux/13 -> Mux4/3
  Mux3/1 -> Data Type Conversion1/1
  BARO_Data/1 -> Bus Selector2/1
  Bus Selector3/4 -> Terminator24/1  "<mag_strength_gps>"
  Mux5/1 -> Terminator1/1  "Δv_b"
  Demux/18 -> Mux2/2
  Mux7/1 -> Terminator22/1, Scope4/1  "v_ekfnew"
  Bus Selector1/3 -> GPS Fusion1/3(meas_vel), Selector1/1  "<states(5:7)>"
  Bus Selector/1 -> Selector/1  "<gps_LLA_rad>"
  Bus Selector1/4 -> GPS Fusion1/4(gps_alt_ref)  "<gps_alt_aef>"
  Demux/11 -> Mux4/1
  Mux6/1 -> Data Type Conversion5/1, Terminator23/1  "p_ekfnew"
  Switch2/1 -> Delay1/1
  Demux/8 -> Mux6/1  "x_ekfnew"
  Selector1/1 -> Zero-Order Hold9/1
  Demux/5 -> Mux7/1  "vx_ekfnew"
  Demux/17 -> Mux2/1
  Demux/12 -> Mux4/2
  Demux/21 -> Mux1/2
  Bus Selector2/2 -> GPS Fusion1/6(baro_hgt_offset)  "<init_barohgt>"
  Demux/7 -> Mux7/3  "vz_ekfnew"
  Demux/15 -> Mux5/2
  Demux/22 -> Mux1/3
  Demux/1 -> Mux3/1
  Demux/3 -> Mux3/3
  Mag_sensordta/1 -> Bus Selector3/1
  Demux/24 -> Terminator9/1
  Zero-Order Hold9/1 -> Detect Change/1
  Selector/1 -> Data Type Conversion3/1
  Demux/4 -> Mux3/4
  Demux/6 -> Mux7/2  "vy_ekfnew"
  Demux/23 -> Terminator8/1
  Bus Selector2/1 -> GPS Fusion1/5(meas_Hgt)  "<Baro_hgt>"
  GPS Fusion1/1(states) -> Switch1/1
  Bus Selector3/2 -> Data Type Conversion4/1  "<mag_declination_gps>"
  Radians to Degrees/1 -> ekf_new/1  "ekf_new"
  init_states/1 -> Reshape/1
  imu_delta_vel/1 -> Subsystem2/2(imu_delta_vel)
  imu_delta_angle/1 -> Subsystem2/1(imu_delta_angle)
  Mag Fusion/1(flag) -> Data Type Conversion6/1
  Data Type Conversion5/1 -> p_ekfnew/1
  Data Type Conversion1/1 -> Quaternions to Rotation Angles/1
  Data Type Conversion2/1 -> GPS_xyz/1

== system AFCToolbox2023a/基础导航算法模型库/ECL EKF/Subsystem1 ==
  Gps_sts : Inport
  In2 : Inport  Port=2
  Compare To Constant1 : simulink/Logic and Bit Operations/Compare To Constant  relop=>=  const=3  OutDataTypeStr=boolean
  Compare To Constant2 : simulink/Logic and Bit Operations/Compare To Constant  relop=>=  const=static_tim  OutDataTypeStr=boolean
  Data Type Conversion1 : DataTypeConversion  OutDataTypeStr=double  SaturateOnIntegerOverflow=off  RndMeth=Floor
  Data Type Conversion2 : DataTypeConversion  OutDataTypeStr=double  SaturateOnIntegerOverflow=off  RndMeth=Floor
  Logical Operator : Logic  AllPortsSameDT=off  OutDataTypeStr=boolean
  enable : Outport
  wires:
  Logical Operator/1 -> enable/1
  Data Type Conversion2/1 -> Logical Operator/2
  Compare To Constant2/1 -> Data Type Conversion2/1
  In2/1 -> Compare To Constant2/1
  Data Type Conversion1/1 -> Logical Operator/1
  Gps_sts/1 -> Compare To Constant1/1
  Compare To Constant1/1 -> Data Type Conversion1/1

== system AFCToolbox2023a/基础导航算法模型库/ECL EKF/Subsystem2 ==
  Gps_sts : Inport
  Tim : Inport  Port=2
  Compare To Constant1 : simulink/Logic and Bit Operations/Compare To Constant  relop=>=  const=3  OutDataTypeStr=boolean
  Compare To Constant2 : simulink/Logic and Bit Operations/Compare To Constant  relop=>=  const=inial_tim  OutDataTypeStr=boolean
  Data Type Conversion1 : DataTypeConversion  OutDataTypeStr=double  SaturateOnIntegerOverflow=off  RndMeth=Floor
  Data Type Conversion2 : DataTypeConversion  OutDataTypeStr=double  SaturateOnIntegerOverflow=off  RndMeth=Floor
  Logical Operator : Logic  AllPortsSameDT=off  OutDataTypeStr=boolean
  enable : Outport
  wires:
  Logical Operator/1 -> enable/1
  Data Type Conversion2/1 -> Logical Operator/2
  Tim/1 -> Compare To Constant2/1
  Compare To Constant2/1 -> Data Type Conversion2/1
  Data Type Conversion1/1 -> Logical Operator/1
  Gps_sts/1 -> Compare To Constant1/1
  Compare To Constant1/1 -> Data Type Conversion1/1

== system AFCToolbox2023a/基础导航算法模型库/ECL EKF/init_state ==
  note: EKF2.cpp -> update() ->
      | ~ ekf.cpp -> initialiseFilter(...) ->
  imu_delta_ang : Inport
  imu_data_del_vel : Inport  Port=2
  gps_LLA_rad : Inport  Port=3
  GPS_Vecef_m/s : Inport  Port=4
  GPSfixtype : Inport  Port=5
  QGC_sensor_reinit : Inport  Port=6
  baro_data_p : Inport  Port=7
  mag : Inport  Port=8
  states : Inport  Port=9
  ALIGN TILT 1 : Subsystem
  Bus Creator3 : BusCreator  Inputs=5
  Bus Selector : BusSelector  OutputSignals=mag_declination_gps
  Display : Display
  InitState_accel1 : Subsystem
  InitState_baro1 : Subsystem
  LLA2NED : Subsystem
  MATLAB Function1 : MATLAB Function  TreatAsAtomicUnit=on
  Math Function2 : Math  Operator=transpose  SignedPower=on
  Product : Product  Multiplication=Matrix(*)
  Quaternions to Direction Cosine Matrix : sharedtransform/Quaternions to  Direction Cosine Matrix  aMode=aMode
      settings: LibrarySourceBlock=|
      | aerolibtransform2/Quaternions to
      | Direction Cosine Matrix
  Scope{,1..3,5} (5 alike) : Scope
  State_mag1 : Subsystem
  states(1:4) : Outport
  states(5:7) : Outport  Port=2
  states(8:10) : Outport  Port=3
  states(17:19) : Outport  Port=4
  BARO_Data : Outport  Port=5
  Mag_sensordata : Outport  Port=6
  GPS_sensordata : Outport  Port=7
  wires:
  MATLAB Function1/3(euler) -> Scope5/1
  MATLAB Function1/1(yaw) -> Scope3/1
  InitState_baro1/1(BARO_Data) -> BARO_Data/1
  InitState_accel1/1(initaccel) -> ALIGN TILT 1/1(initAccel)
  ALIGN TILT 1/1(state(1:4)) -> MATLAB Function1/1("quat "), Display/1
  Product/1 -> states(17:19)/1
  Quaternions to Direction Cosine Matrix/1 -> Math Function2/1
  QGC_sensor_reinit/1 -> LLA2NED/4(QGC_sensor_reinit), InitState_baro1/3(QGC_sensor_reinit)
  GPSfixtype/1 -> LLA2NED/2(GPSfixtype), Bus Creator3/4  "GPSfixtype"
  GPS_Vecef_m/s/1 -> LLA2NED/3(GPS_Vecef_m/s)
  gps_LLA_rad/1 -> LLA2NED/1(gps_LLA_rad), State_mag1/2(gps_LLA_rad), Bus Creator3/3  "gps_LLA_rad"
  mag/1 -> State_mag1/1(mag)  "mag_Body"
  imu_data_del_vel/1 -> InitState_accel1/1(imu_data_del_vel)
  LLA2NED/1(gpsvNEDout) -> Bus Creator3/1, states(5:7)/1, Scope2/1  "states(5:7)"
  LLA2NED/2("gpsposNEDout ") -> Scope1/1, Bus Creator3/2, states(8:10)/1  "states(8:10)"
  Bus Creator3/1 -> GPS_sensordata/1
  states/1 -> InitState_baro1/2(states), State_mag1/3(states)
  State_mag1/2(magdata) -> Bus Selector/1, Mag_sensordata/1
  baro_data_p/1 -> InitState_baro1/1(baro_data_Pa)
  imu_delta_ang/1 -> InitState_baro1/4(imu_delta_ang)
  LLA2NED/3(gps_alt_aef) -> Bus Creator3/5  "gps_alt_aef"
  State_mag1/1(init_MagB) -> Scope/1, MATLAB Function1/2(magMea), Product/2
  Math Function2/1 -> Product/1  "DCM_BO"
  MATLAB Function1/2(quat) -> states(1:4)/1, Quaternions to Direction Cosine Matrix/1
  Bus Selector/1 -> ?  "<mag_declination_gps>"

== system AFCToolbox2023a/ServoCardModule/XSimUnPack/Subsystem2/Subsystem ==
  In1 : Inport
  Enable : EnablePort
  Byte Unpack1 : etargetslib/Byte Unpack  dimensions={7}  datatypes={'single'}  byteAlign=1
      settings: LibrarySourceBlock=embeddedtargetslib/Host Communication/Byte Unpack
  Out1 : Outport
  wires:
  Byte Unpack1/1 -> Out1/1
  In1/1 -> Byte Unpack1/1

== system AFCToolbox2023a/ServoCardModule/XSrvoCmd/设置四个舵机位置与速度指令/GetCheckSum2 ==
  In1 : Inport
  Bitwise AND4 : simulink/Logic and Bit Operations/Bitwise Operator  logicop=AND  UseBitMask=on  BitMask=hex2dec('FF')  BitMaskRealWorld=Stored Integer
      settings: LibrarySourceBlock=|
      | simulink/Quick Insert/Logic and Bit
      | Operations/Bitwise AND
  Bitwise NOT : simulink/Logic and Bit Operations/Bitwise Operator  logicop=NOT  UseBitMask=off  BitMask=bin2dec('11011001')  BitMaskRealWorld=Stored Integer
      settings: LibrarySourceBlock=|
      | simulink/Quick Insert/Logic and Bit
      | Operations/Bitwise NOT
  Data Type Conversion8 : DataTypeConversion  OutDataTypeStr=uint32  SaturateOnIntegerOverflow=off  RndMeth=Floor
  Data Type Conversion9 : DataTypeConversion  OutDataTypeStr=uint8  SaturateOnIntegerOverflow=off  RndMeth=Floor
  Demux1 : Demux  Outputs=[2,-1]
  Sum ofElements4 : Sum  Inputs=+
  Terminator : Terminator
  Out1 : Outport
  wires:
  Data Type Conversion9/1 -> Bitwise NOT/1
  Data Type Conversion8/1 -> Sum ofElements4/1
  Sum ofElements4/1 -> Bitwise AND4/1
  Bitwise AND4/1 -> Data Type Conversion9/1
  Demux1/2 -> Data Type Conversion8/1
  Demux1/1 -> Terminator/1
  In1/1 -> Demux1/1
  Bitwise NOT/1 -> Out1/1

== system AFCToolbox2023a/ServoCardModule/XSrvoCmd/设置四个舵机位置与速度指令/Subsystem1 ==
  p : Inport
  Byte Pack : etargetslib/Byte Pack  datatypes={'uint8','uint16','uint16','uint16'}  byteAlign=1
  Constant : Constant  Value=id
  Constant11 : Constant  Value=3000
  Constant3 : Constant  Value=360/4096  OutDataTypeStr=double
  Data Type Conversion4 : DataTypeConversion  OutDataTypeStr=uint16  SaturateOnIntegerOverflow=off  RndMeth=Floor
  Data Type Conversion5 : DataTypeConversion  OutDataTypeStr=uint8  SaturateOnIntegerOverflow=off  RndMeth=Floor
  Data Type Conversion6 : DataTypeConversion  OutDataTypeStr=uint16  SaturateOnIntegerOverflow=off  RndMeth=Floor
  Divide3 : Product  Inputs=*/
  time : Constant  Value=0  OutDataTypeStr=uint16
  Out1 : Outport
  wires:
  Byte Pack/1 -> Out1/1
  Constant/1 -> Data Type Conversion5/1
  p/1 -> Divide3/1
  Data Type Conversion5/1 -> Byte Pack/1
  time/1 -> Byte Pack/3
  Constant11/1 -> Data Type Conversion6/1
  Data Type Conversion4/1 -> Byte Pack/2
  Constant3/1 -> Divide3/2
  Data Type Conversion6/1 -> Byte Pack/4
  Divide3/1 -> Data Type Conversion4/1

== system AFCToolbox2023a/ServoCardModule/XSrvoCmd/设置四个舵机位置与速度指令/Subsystem2 ==
  p : Inport
  Byte Pack : etargetslib/Byte Pack  datatypes={'uint8','uint16','uint16','uint16'}  byteAlign=1
  Constant : Constant  Value=id
  Constant11 : Constant  Value=3000
  Constant3 : Constant  Value=360/4096  OutDataTypeStr=double
  Data Type Conversion4 : DataTypeConversion  OutDataTypeStr=uint16  SaturateOnIntegerOverflow=off  RndMeth=Floor
  Data Type Conversion5 : DataTypeConversion  OutDataTypeStr=uint8  SaturateOnIntegerOverflow=off  RndMeth=Floor
  Data Type Conversion6 : DataTypeConversion  OutDataTypeStr=uint16  SaturateOnIntegerOverflow=off  RndMeth=Floor
  Divide3 : Product  Inputs=*/
  time : Constant  Value=0  OutDataTypeStr=uint16
  Out1 : Outport
  wires:
  Divide3/1 -> Data Type Conversion4/1
  Data Type Conversion6/1 -> Byte Pack/4
  Constant3/1 -> Divide3/2
  Data Type Conversion4/1 -> Byte Pack/2
  time/1 -> Byte Pack/3
  Data Type Conversion5/1 -> Byte Pack/1
  p/1 -> Divide3/1
  Constant/1 -> Data Type Conversion5/1
  Byte Pack/1 -> Out1/1
  Constant11/1 -> Data Type Conversion6/1

== system AFCToolbox2023a/ServoCardModule/XSrvoCmd/设置四个舵机位置与速度指令/Subsystem3 ==
  p : Inport
  Byte Pack : etargetslib/Byte Pack  datatypes={'uint8','uint16','uint16','uint16'}  byteAlign=1
  Constant : Constant  Value=id
  Constant11 : Constant  Value=3000
  Constant3 : Constant  Value=360/4096  OutDataTypeStr=double
  Data Type Conversion4 : DataTypeConversion  OutDataTypeStr=uint16  SaturateOnIntegerOverflow=off  RndMeth=Floor
  Data Type Conversion5 : DataTypeConversion  OutDataTypeStr=uint8  SaturateOnIntegerOverflow=off  RndMeth=Floor
  Data Type Conversion6 : DataTypeConversion  OutDataTypeStr=uint16  SaturateOnIntegerOverflow=off  RndMeth=Floor
  Divide3 : Product  Inputs=*/
  time : Constant  Value=0  OutDataTypeStr=uint16
  Out1 : Outport
  wires:
  Byte Pack/1 -> Out1/1
  Constant/1 -> Data Type Conversion5/1
  p/1 -> Divide3/1
  Data Type Conversion5/1 -> Byte Pack/1
  time/1 -> Byte Pack/3
  Data Type Conversion4/1 -> Byte Pack/2
  Constant3/1 -> Divide3/2
  Data Type Conversion6/1 -> Byte Pack/4
  Divide3/1 -> Data Type Conversion4/1
  Constant11/1 -> Data Type Conversion6/1

== system AFCToolbox2023a/ServoCardModule/XSrvoCmd/设置四个舵机位置与速度指令/Subsystem5 ==
  p : Inport
  Byte Pack : etargetslib/Byte Pack  datatypes={'uint8','uint16','uint16','uint16'}  byteAlign=1
  Constant : Constant  Value=id
  Constant11 : Constant  Value=3000
  Constant3 : Constant  Value=360/4096  OutDataTypeStr=double
  Data Type Conversion4 : DataTypeConversion  OutDataTypeStr=uint16  SaturateOnIntegerOverflow=off  RndMeth=Floor
  Data Type Conversion5 : DataTypeConversion  OutDataTypeStr=uint8  SaturateOnIntegerOverflow=off  RndMeth=Floor
  Data Type Conversion6 : DataTypeConversion  OutDataTypeStr=uint16  SaturateOnIntegerOverflow=off  RndMeth=Floor
  Divide3 : Product  Inputs=*/
  time : Constant  Value=0  OutDataTypeStr=uint16
  Out1 : Outport
  wires:
  Divide3/1 -> Data Type Conversion4/1
  Data Type Conversion6/1 -> Byte Pack/4
  Constant3/1 -> Divide3/2
  Data Type Conversion4/1 -> Byte Pack/2
  time/1 -> Byte Pack/3
  Data Type Conversion5/1 -> Byte Pack/1
  p/1 -> Divide3/1
  Constant/1 -> Data Type Conversion5/1
  Byte Pack/1 -> Out1/1
  Constant11/1 -> Data Type Conversion6/1

== system AFCToolbox2023a/ServoCardModule/XSrvoSamp/SrvoPro/Subsystem ==
  In1 : Inport
  Enable : EnablePort
  Byte Unpack22 : etargetslib/Byte Unpack  dimensions={[1]}  datatypes={'int16'}  byteAlign=1
      settings: LibrarySourceBlock=embeddedtargetslib/Host Communication/Byte Unpack
  Constant23 : Constant  Value=360/4096
  Data Type Conversion2 : DataTypeConversion  OutDataTypeStr=double  SaturateOnIntegerOverflow=off  RndMeth=Floor
  Divide24 : Product  Inputs=**
  Outport : Outport
  wires:
  Data Type Conversion2/1 -> Divide24/2
  In1/1 -> Byte Unpack22/1
  Constant23/1 -> Divide24/1
  Byte Unpack22/1 -> Data Type Conversion2/1
  Divide24/1 -> Outport/1

== system AFCToolbox2023a/ServoCardModule/XSrvoSamp/SrvoPro1/Subsystem ==
  In1 : Inport
  Enable : EnablePort
  Byte Unpack22 : etargetslib/Byte Unpack  dimensions={[1]}  datatypes={'int16'}  byteAlign=1
      settings: LibrarySourceBlock=embeddedtargetslib/Host Communication/Byte Unpack
  Constant23 : Constant  Value=360/4096
  Data Type Conversion2 : DataTypeConversion  OutDataTypeStr=double  SaturateOnIntegerOverflow=off  RndMeth=Floor
  Divide24 : Product  Inputs=**
  Outport : Outport
  wires:
  Data Type Conversion2/1 -> Divide24/2
  In1/1 -> Byte Unpack22/1
  Constant23/1 -> Divide24/1
  Byte Unpack22/1 -> Data Type Conversion2/1
  Divide24/1 -> Outport/1

== system AFCToolbox2023a/ServoCardModule/XSrvoSamp/SrvoPro2/Subsystem ==
  In1 : Inport
  Enable : EnablePort
  Byte Unpack22 : etargetslib/Byte Unpack  dimensions={[1]}  datatypes={'int16'}  byteAlign=1
      settings: LibrarySourceBlock=embeddedtargetslib/Host Communication/Byte Unpack
  Constant23 : Constant  Value=360/4096
  Data Type Conversion2 : DataTypeConversion  OutDataTypeStr=double  SaturateOnIntegerOverflow=off  RndMeth=Floor
  Divide24 : Product  Inputs=**
  Outport : Outport
  wires:
  Data Type Conversion2/1 -> Divide24/2
  In1/1 -> Byte Unpack22/1
  Constant23/1 -> Divide24/1
  Byte Unpack22/1 -> Data Type Conversion2/1
  Divide24/1 -> Outport/1

== system AFCToolbox2023a/ServoCardModule/XSrvoSamp/SrvoPro3/Subsystem ==
  In1 : Inport
  Enable : EnablePort
  Byte Unpack22 : etargetslib/Byte Unpack  dimensions={[1]}  datatypes={'int16'}  byteAlign=1
      settings: LibrarySourceBlock=embeddedtargetslib/Host Communication/Byte Unpack
  Constant23 : Constant  Value=360/4096
  Data Type Conversion2 : DataTypeConversion  OutDataTypeStr=double  SaturateOnIntegerOverflow=off  RndMeth=Floor
  Divide24 : Product  Inputs=**
  Outport : Outport
  wires:
  Data Type Conversion2/1 -> Divide24/2
  In1/1 -> Byte Unpack22/1
  Constant23/1 -> Divide24/1
  Byte Unpack22/1 -> Data Type Conversion2/1
  Divide24/1 -> Outport/1

== system AFCToolbox2023a/SimuMoudle/Forces & Moments1/Forces/Subsystem ==
  Zero : Inport
  g0 : Inport  Port=2
  Mux1 : Mux  Inputs=3
  gravity : Outport
  wires:
  Zero/1 -> Mux1/2, Mux1/1
  Mux1/1 -> gravity/1
  g0/1 -> Mux1/3
